simulink model "EE463_Buck_Baslangic"  (R2025b)
settings: Solver=ode23t  StartTime=0  StopTime=0.025000000000000001  MaxStep=1.0869565217391305e-07  RelTol=1e-6  AbsTol=1e-8
model workspace (MAT data in the model file):
  Cval = 0.0001
  DCR = 0.0069
  ESR = 0.01
  Ki = 25
  Kp = 0.003
  Lval = 1e-05
  Rval = 2.4
  Vin0 = 48
  Vin1 = 48
  Vref = 12
  fsw = 230000
  loopOn = 1
  tStep = 0.008
libraries: fl_lib x10, nesl_utility x7, simulink x1
settings Model: Creator=Nskhe  LastModifiedBy=Nskhe

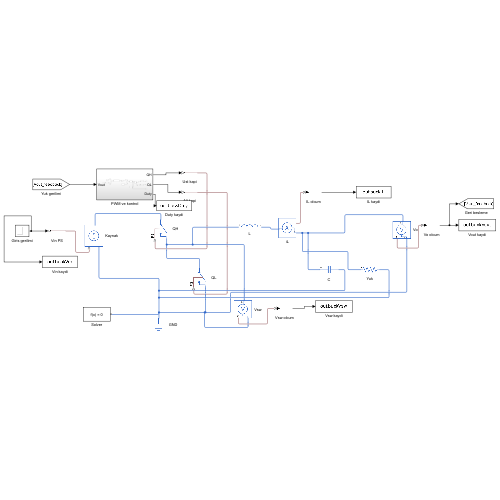
[thumbnail: Simulink's stored preview of the top-level diagram]
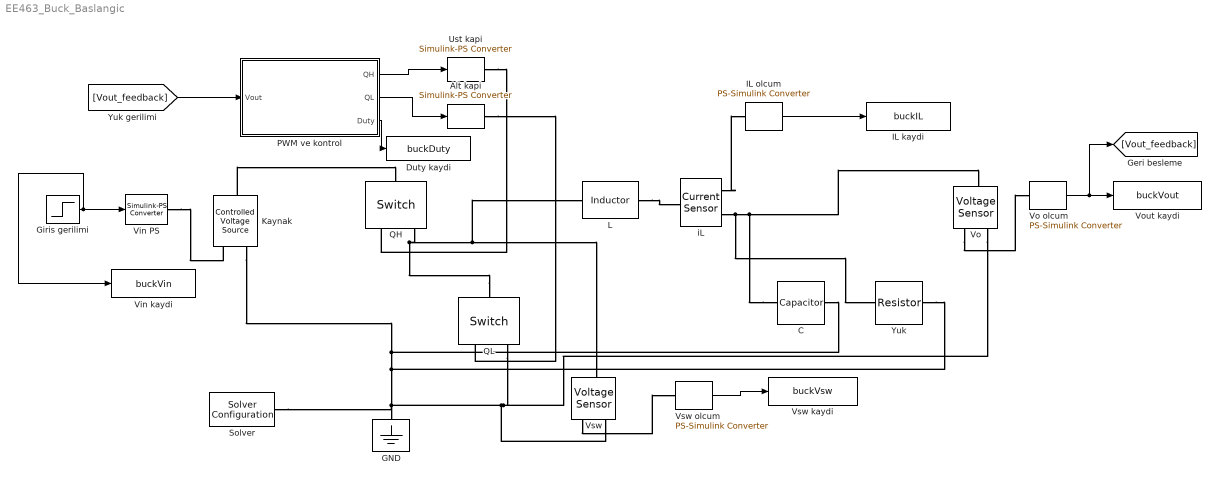
== system EE463_Buck_Baslangic ==
  Alt kapi : nesl_utility/Simulink-PS Converter  PhysicalDomain=network_engine_domain  SubClassName=ps_input  LeftPortType=input  RightPortType=output  PseudoPeriodic=off  Frequencies=[]  NoiseDistribution=none  NoiseParameters=[]  Unit=1  AffineConversion=off  FilteringAndDerivatives=zero  SimscapeFilterOrder=1  InputFilterTimeConstant=0.001  UdotUserProvided=0
  C : fl_lib/Electrical/Electrical Elements/Capacitor  c=Cval F  r=ESR Ohm  g=0 1/Ohm  i_specify=off  i_priority=None  i=0 A  i_nominal_specify=off  i_nominal_value=1  i_nominal_unit=A  v_specify=off  v_priority=None  v=0 V  v_nominal_specify=off  v_nominal_value=1  v_nominal_unit=V  vc_specify=off  vc_priority=High  vc=0 V  vc_nominal_specify=off  vc_nominal_value=1  vc_nominal_unit=V
  Duty kaydi : ToWorkspace  VariableName=buckDuty  SaveFormat=Timeseries  SampleTime=1/fsw
  GND : fl_lib/Electrical/Electrical Elements/Electrical Reference
  Giris gerilimi : Step  Time=tStep  Before=Vin0  After=Vin1  SampleTime=0
  IL kaydi : ToWorkspace  VariableName=buckIL  SaveFormat=Timeseries  SampleTime=-1
  IL olcum : nesl_utility/PS-Simulink Converter  PhysicalDomain=network_engine_domain  SubClassName=ps_output  LeftPortType=input  RightPortType=output  PseudoPeriodic=off  Frequencies=[]  VectorFormat=inherit  Unit=A  AffineConversion=off
  Kaynak : fl_lib/Electrical/Electrical Sources/Controlled Voltage Source
  L : fl_lib/Electrical/Electrical Elements/Inductor  l=Lval H  r=DCR Ohm  g=1e-9 1/Ohm  i_specify=off  i_priority=None  i=0 A  i_nominal_specify=off  i_nominal_value=1  i_nominal_unit=A  v_specify=off  v_priority=None  v=0 V  v_nominal_specify=off  v_nominal_value=1  v_nominal_unit=V  i_L_specify=off  i_L_priority=High  i_L=0 A  i_L_nominal_specify=off  i_L_nominal_value=1  i_L_nominal_unit=A
  PWM ve kontrol : Subsystem
  QH : fl_lib/Electrical/Electrical Elements/Switch  R_closed=0.0052 Ohm  G_open=1e-8 1/Ohm  Threshold=0.5  i_specify=off  i_priority=None  i=0 A  i_nominal_specify=off  i_nominal_value=1  i_nominal_unit=A  v_specify=off  v_priority=None  v=0 V  v_nominal_specify=off  v_nominal_value=1  v_nominal_unit=V
  QL : fl_lib/Electrical/Electrical Elements/Switch  R_closed=0.0052 Ohm  G_open=1e-8 1/Ohm  Threshold=0.5  i_specify=off  i_priority=None  i=0 A  i_nominal_specify=off  i_nominal_value=1  i_nominal_unit=A  v_specify=off  v_priority=None  v=0 V  v_nominal_specify=off  v_nominal_value=1  v_nominal_unit=V
  Solver : nesl_utility/Solver Configuration  PhysicalDomain=network_engine_domain  SubClassName=solver  LeftPortType=input  RightPortType=generic  Tones=[]  Harmonics=[]  SimulateNoise=off  Profile=off  UseLocalSampling=off  EnableSwitchedLinearOptims=on  FrequencyDomain=off  UseCCode=off  RelTol=0.001  AbsTol=0.001  MinStep=1e-09  ToWorkspace=off  RevertToSquareIcSolve=off  NumHomotopyIterations=100  PhasorMode=off  PhasorModeNumHarmonics=1  ConsistencySolver=NEWTON_XTOL_AFTER_FTOL  IndexReductionMethod=DerivativeReplacement  DoDC=off  ResidualTolerance=1e-09  ConsistencyTolSource=GLOBAL  ConsistencyAbsTol=0.001  ConsistencyRelTol=0.001  ConsistencyTolFactor=0.001  UseLocalSolver=off  LocalSolverChoice=NE_BACKWARD_EULER_ADVANCER  ResolveIndetEquations=on  FunctionEvalNumThread=1  LocalSolverSampleTime=0.001  DoFixedCost=off  MaxNonlinIter=3  MaxModeIter=2  ComputeImpulses=off  ImpulseIterations=2  LinearAlgebra=auto  LinearAlgebraNumThread=0  EquationFormulation=NE_TIME_EF  DelaysMemoryBudget=1024  AutomaticFiltering=on  FilteringTimeConstant=0.001  PartitionStorageMethod=AS_NEEDED  PartitionMemoryBudget=1024  PartitionMethod=ROBUST  MultibodyUseLocalSolver=off  MultibodyLocalSolverChoice=ODE1  MultibodyLocalSolverSampleTime=0.001
  Ust kapi : nesl_utility/Simulink-PS Converter  PhysicalDomain=network_engine_domain  SubClassName=ps_input  LeftPortType=input  RightPortType=output  PseudoPeriodic=off  Frequencies=[]  NoiseDistribution=none  NoiseParameters=[]  Unit=1  AffineConversion=off  FilteringAndDerivatives=zero  SimscapeFilterOrder=1  InputFilterTimeConstant=0.001  UdotUserProvided=0
  Vin PS : nesl_utility/Simulink-PS Converter  PhysicalDomain=network_engine_domain  SubClassName=ps_input  LeftPortType=input  RightPortType=output  PseudoPeriodic=off  Frequencies=[]  NoiseDistribution=none  NoiseParameters=[]  Unit=V  AffineConversion=off  FilteringAndDerivatives=zero  SimscapeFilterOrder=1  InputFilterTimeConstant=0.001  UdotUserProvided=0
  Vin kaydi : ToWorkspace  VariableName=buckVin  SaveFormat=Timeseries  SampleTime=1/fsw
  Vo : fl_lib/Electrical/Electrical Sensors/Voltage Sensor
  Vo olcum : nesl_utility/PS-Simulink Converter  PhysicalDomain=network_engine_domain  SubClassName=ps_output  LeftPortType=input  RightPortType=output  PseudoPeriodic=off  Frequencies=[]  VectorFormat=inherit  Unit=V  AffineConversion=off
  Vout kaydi : ToWorkspace  VariableName=buckVout  SaveFormat=Timeseries  SampleTime=-1
  Vsw : fl_lib/Electrical/Electrical Sensors/Voltage Sensor
  Vsw kaydi : ToWorkspace  VariableName=buckVsw  SaveFormat=Timeseries  SampleTime=-1
  Vsw olcum : nesl_utility/PS-Simulink Converter  PhysicalDomain=network_engine_domain  SubClassName=ps_output  LeftPortType=input  RightPortType=output  PseudoPeriodic=off  Frequencies=[]  VectorFormat=inherit  Unit=V  AffineConversion=off
  Yuk : fl_lib/Electrical/Electrical Elements/Resistor  R=Rval Ohm  i_specify=off  i_priority=None  i=0 A  i_nominal_specify=off  i_nominal_value=1  i_nominal_unit=A  v_specify=off  v_priority=None  v=0 V  v_nominal_specify=off  v_nominal_value=1  v_nominal_unit=V
  iL : fl_lib/Electrical/Electrical Sensors/Current Sensor
  wires:
  Giris gerilimi/1 -> Vin PS/1, Vin kaydi/1
  [Vout_feedback] -> PWM ve kontrol/1(Vout)
  PWM ve kontrol/1(QH) -> Ust kapi/1
  PWM ve kontrol/2(QL) -> Alt kapi/1
  PWM ve kontrol/3(Duty) -> Duty kaydi/1
  Vo olcum/1 -> [Vout_feedback], Vout kaydi/1
  IL olcum/1 -> IL kaydi/1
  Vsw olcum/1 -> Vsw kaydi/1
  connections:
  Vin PS/RConn1 -- Kaynak/RConn1
  Ust kapi/RConn1 -- QH/RConn1
  Alt kapi/RConn1 -- QL/RConn1
  Kaynak/LConn1 -- QH/LConn1
  QL/LConn1 -- L/LConn1 -- Vsw/LConn1 -- QH/RConn2
  L/RConn1 -- iL/LConn1
  C/LConn1 -- iL/RConn2 -- Yuk/LConn1 -- Vo/LConn1
  Kaynak/RConn2 -- Vo/RConn2 -- QL/RConn2 -- Vsw/RConn2 -- GND/LConn1 -- Solver/RConn1 -- Yuk/RConn1 -- C/RConn1
  iL/RConn1 -- IL olcum/LConn1
  Vo/RConn1 -- Vo olcum/LConn1
  Vsw/RConn1 -- Vsw olcum/LConn1

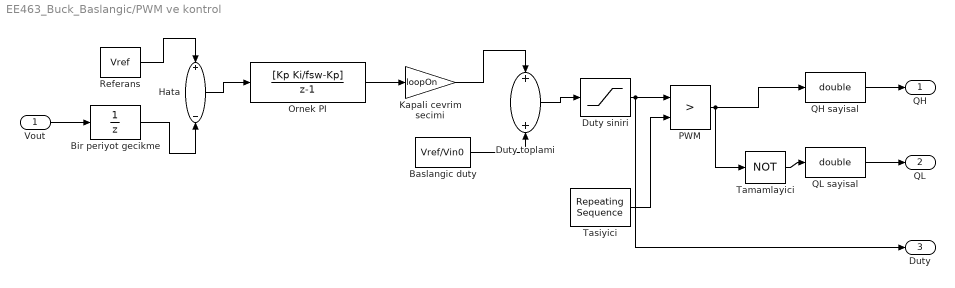
== system EE463_Buck_Baslangic/PWM ve kontrol ==
  Vout : Inport
  Baslangic duty : Constant  Value=Vref/Vin0
  Bir periyot gecikme : UnitDelay  InitialCondition=Vref  SampleTime=1/fsw  HasFrameUpgradeWarning=on
  Duty siniri : Saturate  UpperLimit=0.95  LowerLimit=0.05
  Duty toplami : Sum
  Hata : Sum  Inputs=+-
  Kapali cevrim secimi : Gain  Gain=loopOn
  Ornek PI : DiscreteTransferFcn  Numerator=[Kp Ki/fsw-Kp]  Denominator=[1 -1]  SampleTime=1/fsw
  PWM : RelationalOperator  Operator=>
  QH sayisal : DataTypeConversion  OutDataTypeStr=double  SaturateOnIntegerOverflow=off  RndMeth=Floor
  QL sayisal : DataTypeConversion  OutDataTypeStr=double  SaturateOnIntegerOverflow=off  RndMeth=Floor
  Referans : Constant  Value=Vref
  Tamamlayici : Logic  Operator=NOT
  Tasiyici : simulink/Sources/Repeating Sequence  rep_seq_t=[0 1/fsw]  rep_seq_y=[0 1]
  QH : Outport
  QL : Outport  Port=2
  Duty : Outport  Port=3
  wires:
  Vout/1 -> Bir periyot gecikme/1
  Referans/1 -> Hata/1
  Bir periyot gecikme/1 -> Hata/2
  Hata/1 -> Ornek PI/1
  Ornek PI/1 -> Kapali cevrim secimi/1
  Kapali cevrim secimi/1 -> Duty toplami/1
  Baslangic duty/1 -> Duty toplami/2
  Duty toplami/1 -> Duty siniri/1
  Duty siniri/1 -> PWM/1, Duty/1
  Tasiyici/1 -> PWM/2
  PWM/1 -> QH sayisal/1, Tamamlayici/1
  Tamamlayici/1 -> QL sayisal/1
  QH sayisal/1 -> QH/1
  QL sayisal/1 -> QL/1
